simulink model "test_afe_uvw_ctrl"  (R2026a)
settings: Solver=FixedStepDiscrete  SolverType=Fixed-step  SolverMode=SingleTasking  StartTime=0.0  StopTime=tb.t_end  FixedStep=tb.ts
undefined symbols (not defined in the file or in its folder): tb
libraries: afe_uvw_ctrl x5
Description:
  | Test bench of library/masked_models/afe_uvw_ctrl: the five blocks (grid_voltage_sequences, frt_vde4110, grid_current_sequences_q_ctrl, current_ctrl_uvw, islanding_detector) in the chain of the model afe_uvw_three_phase, fed by the MATLAB Function test_source (grid voltage with a dip and a frequency ramp, PLL angle, references; afe_uvw_ctrl_test_source.m) and closed on the MATLAB Function rl_plant (three RL branches, afe_uvw_ctrl_test_plant.m) through a Unit Delay; grid current = -stack current. Fixed-step discrete, step tb.ts. Variables p and tb from afe_uvw_ctrl_test_param.m; run and check with afe_uvw_ctrl_test_run.m (it also compares the model with the same functions called in a MATLAB loop). Generated by tools/make_afe_uvw_ctrl.py.
settings Model: Creator=pwr-control  LastModifiedBy=pwr-control
settings DataIOCC: SaveTime=on  SaveFormat=Dataset  ReturnWorkspaceOutputs=on  LimitDataPoints=off

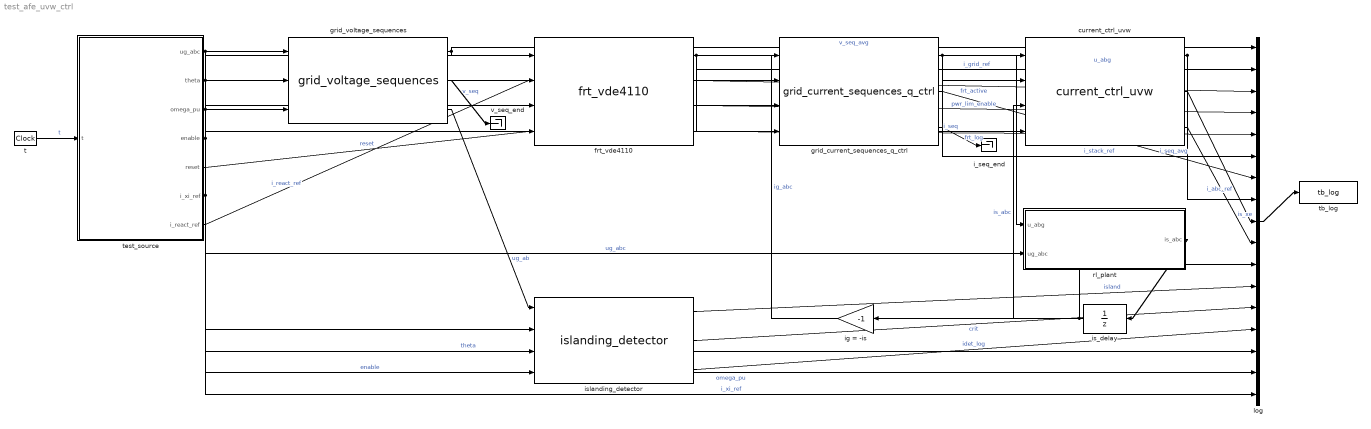
== system test_afe_uvw_ctrl ==
  t : DigitalClock  SampleTime=tb.ts
  test_source : MATLAB Function  TreatAsAtomicUnit=on
  grid_voltage_sequences : afe_uvw_ctrl/grid_voltage_sequences  p=p
  frt_vde4110 : afe_uvw_ctrl/frt_vde4110  p=p
  grid_current_sequences_q_ctrl : afe_uvw_ctrl/grid_current_sequences_q_ctrl  p=p
  current_ctrl_uvw : afe_uvw_ctrl/current_ctrl_uvw  p=p
  islanding_detector : afe_uvw_ctrl/islanding_detector  p=p
  rl_plant : MATLAB Function  TreatAsAtomicUnit=on
  is_delay : UnitDelay  InitialCondition=zeros(3, 1)  SampleTime=-1
  ig = -is : Gain  Gain=-1
  log : Mux  Inputs=17
  tb_log : ToWorkspace  VariableName=tb_log  SampleTime=-1  SaveFormat=Array
  v_seq_end : Terminator
  i_seq_end : Terminator
  wires:
  t/1 -> test_source/1(t)  "t"
  test_source/1(ug_abc) -> grid_voltage_sequences/1, rl_plant/2(ug_abc)  "ug_abc"
  test_source/2(theta) -> grid_voltage_sequences/2, grid_current_sequences_q_ctrl/2, current_ctrl_uvw/4, islanding_detector/2, log/15  "theta"
  test_source/3(omega_pu) -> grid_voltage_sequences/3, grid_current_sequences_q_ctrl/3, islanding_detector/3, log/16  "omega_pu"
  test_source/4(enable) -> frt_vde4110/3, islanding_detector/4  "enable"
  test_source/5(reset) -> frt_vde4110/4  "reset"
  test_source/6(i_xi_ref) -> current_ctrl_uvw/1, log/17  "i_xi_ref"
  test_source/7(i_react_ref) -> frt_vde4110/2  "i_react_ref"
  grid_voltage_sequences/1 -> frt_vde4110/1, log/1  "v_seq_avg"
  grid_voltage_sequences/3 -> islanding_detector/1  "ug_ab"
  frt_vde4110/1 -> grid_current_sequences_q_ctrl/4, log/2  "i_grid_ref"
  frt_vde4110/2 -> log/3  "frt_active"
  frt_vde4110/3 -> log/4  "pwr_lim_enable"
  frt_vde4110/4 -> log/5  "frt_log"
  grid_current_sequences_q_ctrl/1 -> current_ctrl_uvw/2, log/6  "i_stack_ref"
  grid_current_sequences_q_ctrl/2 -> log/7  "i_seq_avg"
  current_ctrl_uvw/1 -> rl_plant/1(u_abg), log/8  "u_abg"
  current_ctrl_uvw/2 -> log/9  "i_abc_ref"
  current_ctrl_uvw/3 -> log/10  "is_xe"
  rl_plant/1(is_abc) -> is_delay/1
  is_delay/1 -> current_ctrl_uvw/3, ig = -is/1, log/11  "is_abc"
  ig = -is/1 -> grid_current_sequences_q_ctrl/1  "ig_abc"
  islanding_detector/1 -> log/12  "island"
  islanding_detector/2 -> log/13  "crit"
  islanding_detector/3 -> log/14  "idet_log"
  log/1 -> tb_log/1
  grid_voltage_sequences/2 -> v_seq_end/1  "v_seq"
  grid_current_sequences_q_ctrl/3 -> i_seq_end/1  "i_seq"

== matlab function test_afe_uvw_ctrl/test_source ==
  data: t input size=1; ug_abc output size=[3 1]; theta output size=1; omega_pu output size=1; enable output size=1; reset output size=1; i_xi_ref output size=1; i_react_ref output size=[2 1]; tb parameter
function [ug_abc, theta, omega_pu, enable, reset, i_xi_ref, i_react_ref] = afe_uvw_ctrl_test_source(t, tb)
%AFE_UVW_CTRL_TEST_SOURCE  Grid voltage, PLL angle and references of the test bench, closed form of the time.
%
%   [ug_abc, theta, omega_pu, enable, reset, i_xi_ref, i_react_ref] = afe_uvw_ctrl_test_source(t, tb)
%
%   MATLAB Function of test_afe_uvw_ctrl.slx (and of afe_uvw_ctrl_test_loop.m). The grid is an ideal
%   source: positive sequence 1 pu (tb.dip_pos during the dip), negative sequence tb.dip_neg during the
%   dip, 5th and 7th harmonics, frequency tb.f_pu until tb.t_drift and then a ramp of tb.df_pu_dt
%   capped at tb.f_pu_max. theta is the angle of the positive sequence, as an ideal PLL would give it,
%   omega_pu its pulsation in pu. No states: everything is a function of t.
%
%   Outputs  ug_abc [3x1] pu, theta [rad] in [0, 2 pi), omega_pu [pu], enable and reset (0/1) for
%   frt_vde4110 (enable also for islanding_detector), i_xi_ref [pu], i_react_ref [2x1] [pos; neg] pu.
%
%   See also afe_uvw_ctrl_test_param, afe_uvw_ctrl_test_plant.

    % ---- frequency and angle
    if t <= tb.t_drift
        omega_pu = tb.f_pu;
        th = tb.f_pu*t;
    else
        tau = t - tb.t_drift;
        tau_cap = (tb.f_pu_max - tb.f_pu)/tb.df_pu_dt;          % the ramp reaches the cap after this time
        if tau <= tau_cap
            omega_pu = tb.f_pu + tb.df_pu_dt*tau;
            th = tb.f_pu*t + 0.5*tb.df_pu_dt*tau^2;
        else
            omega_pu = tb.f_pu_max;
            th = tb.f_pu*(tb.t_drift + tau_cap) + 0.5*tb.df_pu_dt*tau_cap^2 + tb.f_pu_max*(tau - tau_cap);
        end
    end
    theta = mod(tb.omega_nom*th, 2*pi);

    % ---- voltage: sequences and harmonics in alpha/beta, then abc (amplitude-invariant Clarke)
    if t >= tb.t_dip(1) && t < tb.t_dip(2)
        vp = tb.dip_pos;
        vn = tb.dip_neg;
    else
        vp = 1;
        vn = 0;
    end
    ua = vp*cos(theta) + vn*cos(-theta + tb.dip_neg_phase) ...
         + tb.h7*cos(7*theta + tb.h7_phase) + tb.h5*cos(-5*theta + tb.h5_phase);
    ub = vp*sin(theta) + vn*sin(-theta + tb.dip_neg_phase) ...
         + tb.h7*sin(7*theta + tb.h7_phase) + tb.h5*sin(-5*theta + tb.h5_phase);
    ug_abc = [ua; -0.5*ua + sqrt(3)/2*ub; -0.5*ua - sqrt(3)/2*ub];

    % ---- enables and references
    enable = double(t >= tb.t_enable);
    reset = double(t < tb.t_reset);
    i_xi_ref = tb.i_xi_ref*double(t >= tb.t_ctrl_on);
    i_react_ref = [tb.i_react_pos; tb.i_react_neg]*double(t >= tb.t_react);
end

== matlab function test_afe_uvw_ctrl/rl_plant ==
  data: u_abg input size=[3 1]; ug_abc input size=[3 1]; is_abc output size=[3 1]; tb parameter
function is_abc = afe_uvw_ctrl_test_plant(u_abg, ug_abc, tb)
%AFE_UVW_CTRL_TEST_PLANT  Three RL branches between the converter and the grid (pu), one step of tb.ts.
%
%   is_abc = afe_uvw_ctrl_test_plant(u_abg, ug_abc, tb)
%
%   MATLAB Function of test_afe_uvw_ctrl.slx (and of afe_uvw_ctrl_test_loop.m). The converter phase
%   voltages are the inverse Clarke transform of [u_alpha; u_beta] plus u_gamma (the zero sequence,
%   the same on the three phases) plus tb.k_ff times the measured grid voltage (the feed-forward of
%   a modulator). Each branch:
%       di/dt = omega_nom/x_l*(u - u_grid - r*i),   u_grid = ug_abc + tb.u0_dc
%   (the DC offset is in the branch voltage, not in the measurement, so the zero-sequence current
%   controller has to cancel it). The step is integrated exactly (voltages held during the step) and
%   the output is the current at the end of the step: the Unit Delay of the bench gives it to the
%   control at the next step, as a measurement taken at the start of the period.
%
%   State (persistent): i [3x1] branch currents [pu].
%
%   See also afe_uvw_ctrl_test_param, afe_uvw_ctrl_test_source.

    persistent i
    if isempty(i)
        i = zeros(3, 1);
    end
    u_abc = [u_abg(1); -0.5*u_abg(1) + sqrt(3)/2*u_abg(2); -0.5*u_abg(1) - sqrt(3)/2*u_abg(2)] ...
            + u_abg(3) + tb.k_ff*ug_abc;
    u_grid = ug_abc + tb.u0_dc;
    a = tb.r*tb.omega_nom/tb.x_l;                           % [1/s] pole of the branch
    e = exp(-a*tb.ts);
    i = e*i + (1 - e)/tb.r*(u_abc - u_grid);
    is_abc = i;
end
